simulink model "RC_Link_Sim"  (R2026b)
settings: Solver=VariableStepAuto
undefined symbols (not defined in the file or in its folder): P, Ts
settings Model: Creator=aomar  LastModifiedBy=aomar

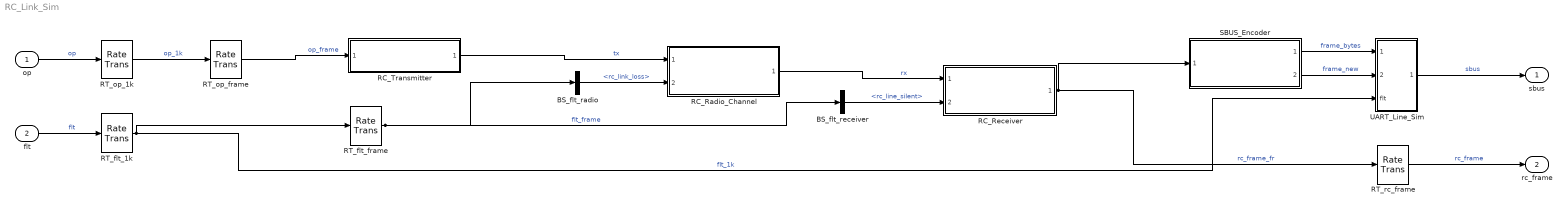
== system RC_Link_Sim ==
  op : Inport  OutDataTypeStr=Bus: Bus_OperatorCmd  SampleTime=Ts.ctrl
  flt : Inport  Port=2  OutDataTypeStr=Bus: Bus_FaultInject  SampleTime=Ts.ctrl
  BS_flt_radio : BusSelector  OutputSignals=rc_link_loss
  BS_flt_receiver : BusSelector  OutputSignals=rc_line_silent
  RC_Radio_Channel : Subsystem  ReferencedSubsystem=rc_radio_channel
  RC_Receiver : Subsystem  ReferencedSubsystem=rc_receiver
  RC_Transmitter : Subsystem  ReferencedSubsystem=rc_transmitter
  RT_flt_1k : RateTransition  InitialCondition=P.ic.Bus_FaultInject  OutPortSampleTime=Ts.base
  RT_flt_frame : RateTransition  InitialCondition=P.ic.Bus_FaultInject  OutPortSampleTime=Ts.rc_frame
  RT_op_1k : RateTransition  InitialCondition=P.ic.Bus_OperatorCmd  OutPortSampleTime=Ts.base
  RT_op_frame : RateTransition  InitialCondition=P.ic.Bus_OperatorCmd  OutPortSampleTime=Ts.rc_frame
  RT_rc_frame : RateTransition  InitialCondition=P.ic.Bus_RcFrame  OutPortSampleTime=Ts.base
  SBUS_Encoder : Subsystem  ReferencedSubsystem=rc_sbus_encoder
  UART_Line_Sim : Subsystem  Description=Contents of subsystems/rc/rc_uart_line_sim.slx, generated by build_rc_link>local_uart_body (inline instead of a nested Subsystem Reference: R2026b Stateflow JIT assertion with a MATLAB Function two Subsystem Reference levels deep).
  sbus : Outport  OutDataTypeStr=Bus: Bus_SbusStream  SampleTime=Ts.base
  rc_frame : Outport  Port=2  OutDataTypeStr=Bus: Bus_RcFrame  SampleTime=Ts.base
  wires:
  op/1 -> RT_op_1k/1  "op"
  flt/1 -> RT_flt_1k/1  "flt"
  RT_op_1k/1 -> RT_op_frame/1  "op_1k"
  RT_flt_1k/1 -> UART_Line_Sim/3(flt), RT_flt_frame/1  "flt_1k"
  RT_op_frame/1 -> RC_Transmitter/1  "op_frame"
  RT_flt_frame/1 -> BS_flt_radio/1, BS_flt_receiver/1  "flt_frame"
  RC_Transmitter/1 -> RC_Radio_Channel/1  "tx"
  BS_flt_radio/1 -> RC_Radio_Channel/2  "<rc_link_loss>"
  RC_Radio_Channel/1 -> RC_Receiver/1  "rx"
  BS_flt_receiver/1 -> RC_Receiver/2  "<rc_line_silent>"
  RC_Receiver/1 -> RT_rc_frame/1, SBUS_Encoder/1  "rc_frame_fr"
  SBUS_Encoder/1 -> UART_Line_Sim/1(frame_bytes)  "frame_bytes"
  SBUS_Encoder/2 -> UART_Line_Sim/2(frame_new)  "frame_new"
  RT_rc_frame/1 -> rc_frame/1  "rc_frame"
  UART_Line_Sim/1(sbus) -> sbus/1  "sbus"

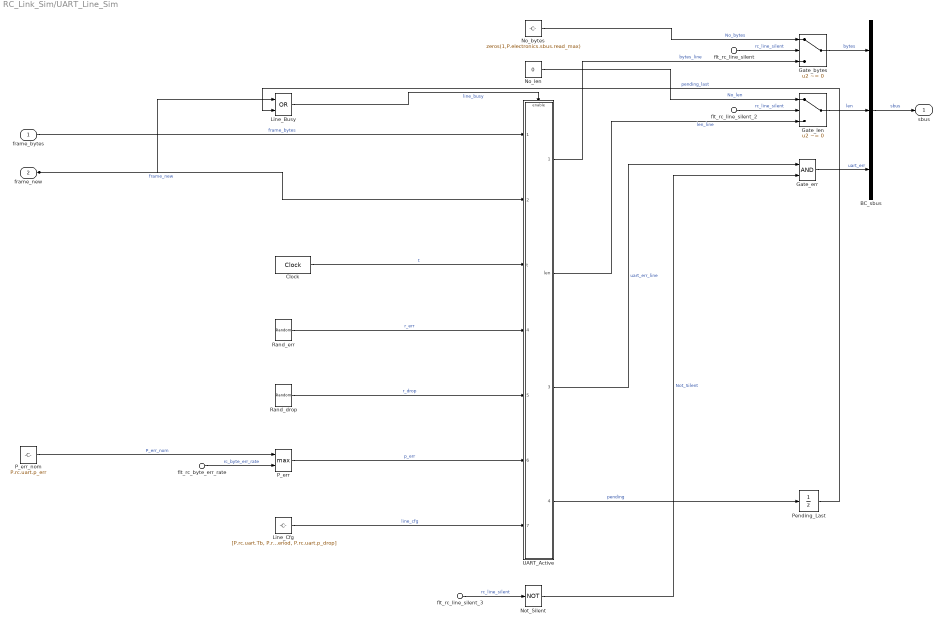
== system RC_Link_Sim/UART_Line_Sim ==
  frame_bytes : Inport  OutDataTypeStr=uint8  PortDimensions=P.electronics.sbus.frame_len  SampleTime=Ts.base
  frame_new : Inport  Port=2  OutDataTypeStr=boolean  PortDimensions=1  SampleTime=Ts.base
  flt_rc_byte_err_rate : Inport  Port=3  PortName=flt  Element=rc_byte_err_rate
  flt_rc_line_silent : Inport  Port=3  PortName=flt  Element=rc_line_silent
  flt_rc_line_silent_2 : Inport  Port=3  PortName=flt  Element=rc_line_silent
  flt_rc_line_silent_3 : Inport  Port=3  PortName=flt  Element=rc_line_silent
  BC_sbus : BusCreator  Inputs=3  OutDataTypeStr=Bus: Bus_SbusStream  NonVirtualBus=on
      settings: InheritFromInputs=off
  Clock : DigitalClock  SampleTime=Ts.base
  Gate_bytes : Switch  Criteria=u2 ~= 0  SaturateOnIntegerOverflow=off  InputSameDT=off
  Gate_err : Logic  AllPortsSameDT=off  OutDataTypeStr=boolean
  Gate_len : Switch  Criteria=u2 ~= 0  SaturateOnIntegerOverflow=off  InputSameDT=off
  Line_Busy : Logic  Operator=OR  AllPortsSameDT=off  OutDataTypeStr=boolean
  Line_Cfg : Constant  Value=[P.rc.uart.Tb, P.rc.uart.phase0, P.rc.uart.drift_ppm, P.rc.frame_period, P.rc.uart.p_drop]  SampleTime=Ts.base
  No_bytes : Constant  Value=zeros(1,P.electronics.sbus.read_max)  OutDataTypeStr=uint8  SampleTime=Ts.base
  No_len : Constant  Value=0  OutDataTypeStr=uint8  SampleTime=Ts.base
  Not_Silent : Logic  Operator=NOT  Inputs=1  AllPortsSameDT=off  OutDataTypeStr=boolean
  P_err : MinMax  Function=max  Inputs=2
  P_err_nom : Constant  Value=P.rc.uart.p_err  SampleTime=Ts.base
  Pending_Last : UnitDelay  SampleTime=Ts.base
  Rand_drop : UniformRandomNumber  Minimum=zeros(1,P.electronics.sbus.frame_len)  Maximum=ones(1,P.electronics.sbus.frame_len)  Seed=P.rc.seed_drop  SampleTime=Ts.base
  Rand_err : UniformRandomNumber  Minimum=zeros(1,P.electronics.sbus.frame_len)  Maximum=ones(1,P.electronics.sbus.frame_len)  Seed=P.rc.seed_err  SampleTime=Ts.base
  UART_Active : Subsystem  Description=Runs sbus_uart_line_sim while a frame is on the line (frame_new OR pending of the previous tick); disabled outputs reset to 0 (no bytes).
  sbus : Outport  OutDataTypeStr=Bus: Bus_SbusStream  SampleTime=Ts.base
  wires:
  frame_bytes/1 -> UART_Active/1(frame)  "frame_bytes"
  frame_new/1 -> Line_Busy/1, UART_Active/2(frame_new)  "frame_new"
  P_err_nom/1 -> P_err/1  "P_err_nom"
  flt_rc_byte_err_rate/1 -> P_err/2  "rc_byte_err_rate"
  Line_Busy/1 -> UART_Active/Enable  "line_busy"
  Rand_err/1 -> UART_Active/4(r_err)  "r_err"
  Rand_drop/1 -> UART_Active/5(r_drop)  "r_drop"
  P_err/1 -> UART_Active/6(p_err)  "p_err"
  Line_Cfg/1 -> UART_Active/7(line_cfg)  "line_cfg"
  Clock/1 -> UART_Active/3(t)  "t"
  flt_rc_line_silent_3/1 -> Not_Silent/1  "rc_line_silent"
  No_bytes/1 -> Gate_bytes/1  "No_bytes"
  No_len/1 -> Gate_len/1  "No_len"
  Not_Silent/1 -> Gate_err/2  "Not_Silent"
  UART_Active/1(bytes) -> Gate_bytes/3  "bytes_line"
  UART_Active/2(len) -> Gate_len/3  "len_line"
  UART_Active/3(uart_err) -> Gate_err/1  "uart_err_line"
  UART_Active/4(pending) -> Pending_Last/1  "pending"
  flt_rc_line_silent/1 -> Gate_bytes/2  "rc_line_silent"
  flt_rc_line_silent_2/1 -> Gate_len/2  "rc_line_silent"
  Gate_err/1 -> BC_sbus/3  "uart_err"
  Pending_Last/1 -> Line_Busy/2  "pending_last"
  Gate_bytes/1 -> BC_sbus/1  "bytes"
  Gate_len/1 -> BC_sbus/2  "len"
  BC_sbus/1 -> sbus/1  "sbus"

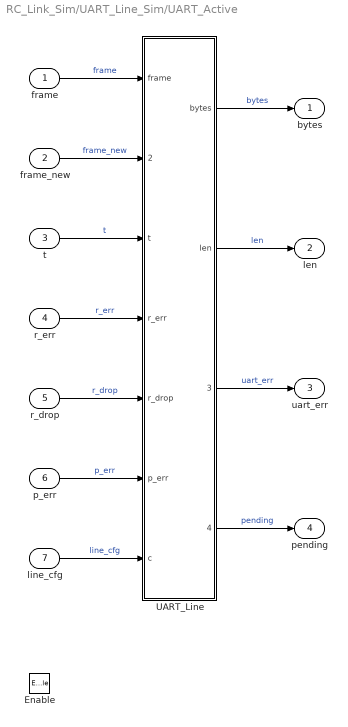
== system RC_Link_Sim/UART_Line_Sim/UART_Active ==
  frame : Inport
  frame_new : Inport  Port=2
  t : Inport  Port=3
  r_err : Inport  Port=4
  r_drop : Inport  Port=5
  p_err : Inport  Port=6
  line_cfg : Inport  Port=7
  Enable : EnablePort
  UART_Line : MATLAB Function  TreatAsAtomicUnit=on
  bytes : Outport  OutputWhenDisabled=reset  InitialOutput=0
  len : Outport  Port=2  OutputWhenDisabled=reset  InitialOutput=0
  uart_err : Outport  Port=3  OutputWhenDisabled=reset  InitialOutput=0
  pending : Outport  Port=4  OutputWhenDisabled=reset  InitialOutput=0
  wires:
  frame/1 -> UART_Line/1(frame)  "frame"
  frame_new/1 -> UART_Line/2(frame_new)  "frame_new"
  t/1 -> UART_Line/3(t)  "t"
  r_err/1 -> UART_Line/4(r_err)  "r_err"
  r_drop/1 -> UART_Line/5(r_drop)  "r_drop"
  p_err/1 -> UART_Line/6(p_err)  "p_err"
  line_cfg/1 -> UART_Line/7(c)  "line_cfg"
  UART_Line/1(bytes) -> bytes/1  "bytes"
  UART_Line/2(len) -> len/1  "len"
  UART_Line/3(uart_err) -> uart_err/1  "uart_err"
  UART_Line/4(pending) -> pending/1  "pending"

== matlab function RC_Link_Sim/UART_Line_Sim/UART_Active/UART_Line ==
  settings: description=SBUS UART byte timing (docs/specs/electronics.md 4.2), simulation only
  data: frame input; bytes output; frame_new input; t input; r_err input; r_drop input; p_err input; c input; len output; uart_err output; pending output
function [bytes, len, uart_err, pending] = fcn(frame, frame_new, t, r_err, r_drop, p_err, c)
%#codegen
% c = [Tb phase0 drift_ppm Tf p_drop] (Constant Line_Cfg)
[bytes, len, uart_err, pending] = sbus_uart_line_sim(frame, frame_new, t, r_err, r_drop, c(1), c(2), c(3), c(4), p_err, c(5));
